simulink model "SVPWM"  (R2018a)
settings: Solver=FixedStepAuto  StartTime=0.0  StopTime=10.0  FixedStep=0.00001  RelTol=1e-3
libraries: simulink x1
settings Model: Creator=18236  LastModifiedBy=18236

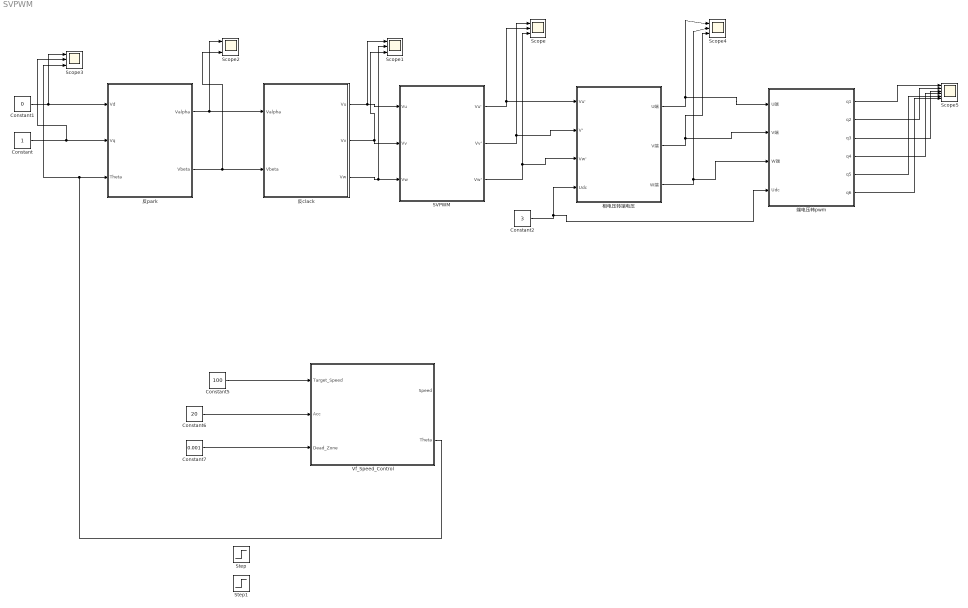
== system SVPWM ==
  Constant : Constant
  Constant1 : Constant  Value=0
  Constant2 : Constant  Value=3
  Constant5 : Constant  Value=100
  Constant6 : Constant  Value=20
  Constant7 : Constant  Value=0.001
  "SVPWM " : Subsystem
  Scope{,1..4} (5 alike) : Scope  NumInputPorts=3
  Scope5 : Scope  NumInputPorts=6
  Step : Step  Time=0  After=50  SampleTime=0
  Step1 : Step  Time=5  After=-100  SampleTime=0
  Vf_Speed_Control : Subsystem
  "反clack " : Subsystem
  "反park " : Subsystem
  "相电压转端电压 " : Subsystem
  端电压转pwm : Subsystem
  wires:
  Constant/1 -> Scope3/2, "反park "/2(Vq)
  Constant1/1 -> Scope3/1, "反park "/1("Vd ")
  "反park "/1("Valpha ") -> Scope2/1, "反clack "/1(Valpha)
  "反park "/2(Vbeta) -> Scope2/3, "反clack "/2(Vbeta)
  "反clack "/1(Vu) -> Scope1/1, "SVPWM "/1("Vu ")
  "反clack "/2(Vv) -> Scope1/3, "SVPWM "/2(Vv)
  "反clack "/3("Vw ") -> Scope1/2, "SVPWM "/3(Vw)
  "SVPWM "/1(Vu') -> "相电压转端电压 "/1(Vu'), Scope/2
  "SVPWM "/2(Vv') -> "相电压转端电压 "/2(V'), Scope/1
  "SVPWM "/3(Vw') -> "相电压转端电压 "/3(Vw'), Scope/3
  Constant2/1 -> 端电压转pwm/4(Udc), "相电压转端电压 "/4(Udc)
  "相电压转端电压 "/1(U端) -> 端电压转pwm/1(U端), Scope4/1
  "相电压转端电压 "/2(V端) -> 端电压转pwm/2(V端), Scope4/3
  "相电压转端电压 "/3(W端) -> 端电压转pwm/3(W端), Scope4/2
  端电压转pwm/1("q1 ") -> Scope5/1
  端电压转pwm/2(q2) -> Scope5/2
  端电压转pwm/3(q3) -> Scope5/3
  端电压转pwm/4(q4) -> Scope5/4
  端电压转pwm/5(q5) -> Scope5/5
  端电压转pwm/6(q6) -> Scope5/6
  Constant5/1 -> Vf_Speed_Control/1(Target_Speed)
  Constant6/1 -> Vf_Speed_Control/2(Acc)
  Constant7/1 -> Vf_Speed_Control/3(Dead_Zone)
  Vf_Speed_Control/2("Theta ") -> "反park "/3("Theta "), Scope3/3

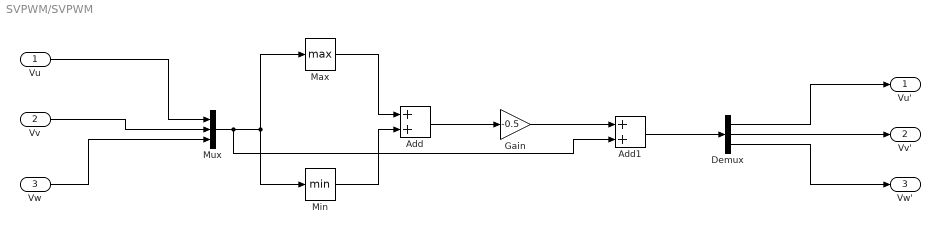
== system SVPWM/SVPWM  ==
  "Vu " : Inport
  Vv : Inport  Port=2
  Vw : Inport  Port=3
  Add : Sum
  Add1 : Sum
  Demux : Demux  Outputs=3
  Gain : Gain  Gain=-0.5
  Max : MinMax  Function=max
  Min : MinMax
  Mux : Mux  Inputs=3
  Vu' : Outport
  Vv' : Outport  Port=2
  Vw' : Outport  Port=3
  wires:
  "Vu "/1 -> Mux/1
  Vv/1 -> Mux/2
  Vw/1 -> Mux/3
  Mux/1 -> Add1/2, Min/1, Max/1
  Max/1 -> Add/1
  Min/1 -> Add/2
  Add/1 -> Gain/1
  Gain/1 -> Add1/1
  Add1/1 -> Demux/1
  Demux/1 -> Vu'/1
  Demux/2 -> Vv'/1
  Demux/3 -> Vw'/1

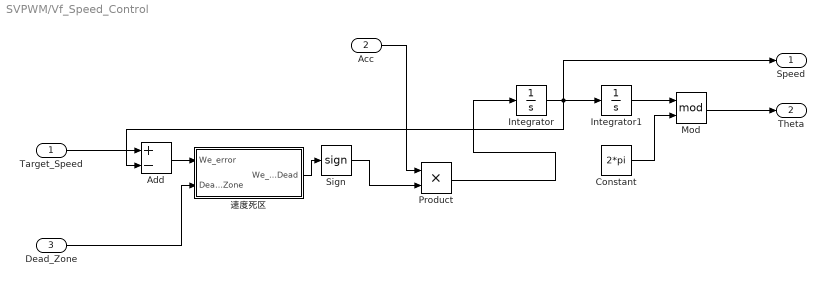
== system SVPWM/Vf_Speed_Control ==
  Target_Speed : Inport
  Acc : Inport  Port=2
  Dead_Zone : Inport  Port=3
  Add : Sum  Inputs=+-
  Constant : Constant  Value=2*pi
  Integrator : Integrator
  Integrator1 : Integrator
  Mod : Math  Operator=mod  SaturateOnIntegerOverflow=on
  Product : Product
  Sign : Signum
  "速度死区 " : MATLAB Function  TreatAsAtomicUnit=on
  Speed : Outport
  "Theta " : Outport  Port=2
  wires:
  Integrator/1 -> Add/2, Speed/1, Integrator1/1
  Integrator1/1 -> Mod/1
  Constant/1 -> Mod/2
  Mod/1 -> "Theta "/1
  Target_Speed/1 -> Add/1
  Add/1 -> "速度死区 "/1(We_error)
  Acc/1 -> Product/1
  Sign/1 -> Product/2
  Product/1 -> Integrator/1
  "速度死区 "/1(We_Error_Dead) -> Sign/1
  Dead_Zone/1 -> "速度死区 "/2(Dead_Zone)

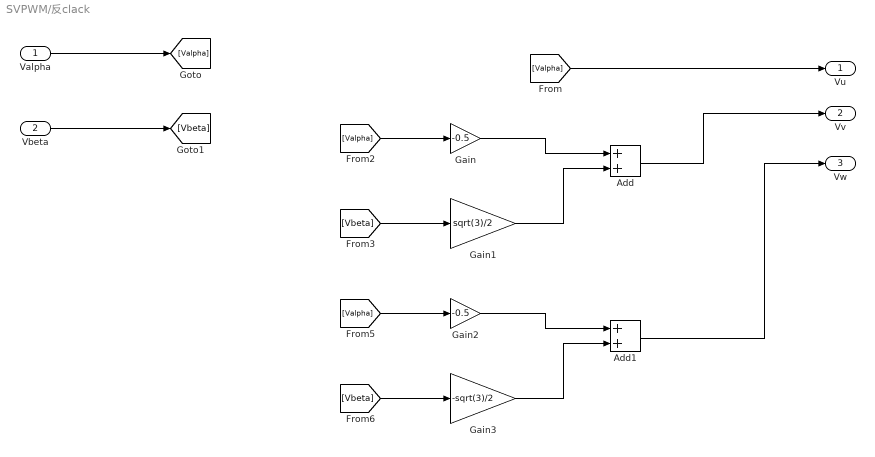
== system SVPWM/反clack  ==
  Valpha : Inport
  Vbeta : Inport  Port=2
  Add : Sum
  Add1 : Sum
  Gain : Gain  Gain=-0.5
  Gain1 : Gain  Gain=sqrt(3)/2
  Gain2 : Gain  Gain=-0.5
  Gain3 : Gain  Gain=-sqrt(3)/2
  Vu : Outport
  Vv : Outport  Port=2
  "Vw " : Outport  Port=3
  wires:
  Valpha/1 -> [Valpha]
  Vbeta/1 -> [Vbeta]
  [Valpha] -> Vu/1
  [Valpha] -> Gain/1
  [Vbeta] -> Gain1/1
  Gain/1 -> Add/1
  Gain1/1 -> Add/2
  Add/1 -> Vv/1
  [Valpha] -> Gain2/1
  [Vbeta] -> Gain3/1
  Gain2/1 -> Add1/1
  Gain3/1 -> Add1/2
  Add1/1 -> "Vw "/1

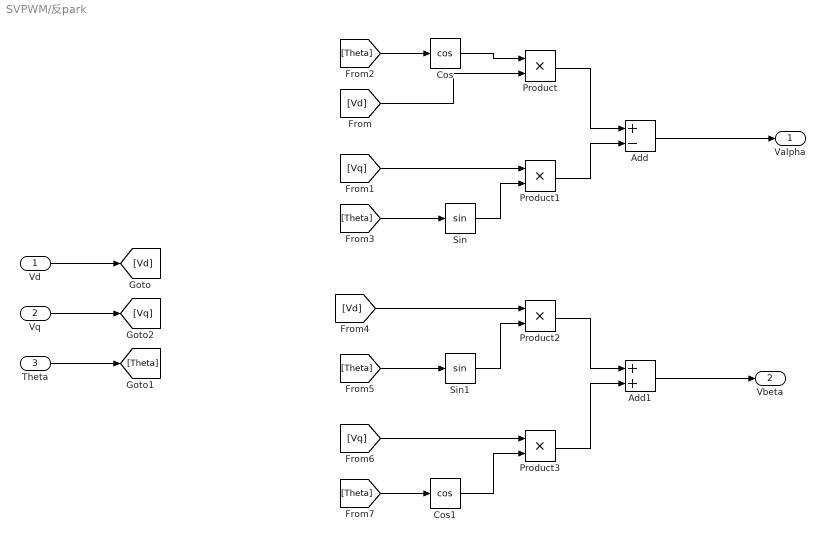
== system SVPWM/反park  ==
  "Vd " : Inport
  Vq : Inport  Port=2
  "Theta " : Inport  Port=3
  Add : Sum  Inputs=+-
  Add1 : Sum
  Cos : Trigonometry  Operator=cos
  Cos1 : Trigonometry  Operator=cos
  Product{,1..3} (4 alike) : Product
  Sin : Trigonometry
  Sin1 : Trigonometry
  "Valpha " : Outport
  Vbeta : Outport  Port=2
  wires:
  "Vd "/1 -> [Vd]
  "Theta "/1 -> [Theta]
  Vq/1 -> [Vq]
  [Theta] -> Cos/1
  Cos/1 -> Product/1
  [Vd] -> Product/2
  [Theta] -> Sin/1
  [Vq] -> Product1/1
  Sin/1 -> Product1/2
  Product/1 -> Add/1
  Product1/1 -> Add/2
  Add/1 -> "Valpha "/1
  [Theta] -> Sin1/1
  [Vd] -> Product2/1
  Sin1/1 -> Product2/2
  [Theta] -> Cos1/1
  [Vq] -> Product3/1
  Cos1/1 -> Product3/2
  Product2/1 -> Add1/1
  Product3/1 -> Add1/2
  Add1/1 -> Vbeta/1

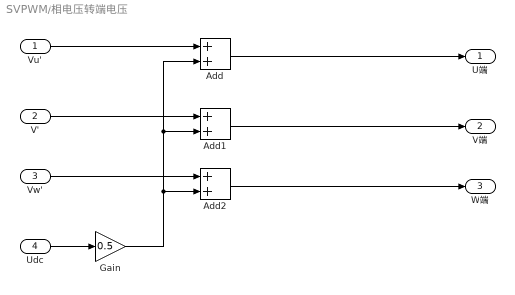
== system SVPWM/相电压转端电压  ==
  Vu' : Inport
  V' : Inport  Port=2
  Vw' : Inport  Port=3
  Udc : Inport  Port=4
  Add : Sum
  Add1 : Sum
  Add2 : Sum
  Gain : Gain  Gain=0.5
  U端 : Outport
  V端 : Outport  Port=2
  W端 : Outport  Port=3
  wires:
  Vu'/1 -> Add/1
  Udc/1 -> Gain/1
  Gain/1 -> Add/2, Add1/2, Add2/2
  Add/1 -> U端/1
  V'/1 -> Add1/1
  Add1/1 -> V端/1
  Vw'/1 -> Add2/1
  Add2/1 -> W端/1

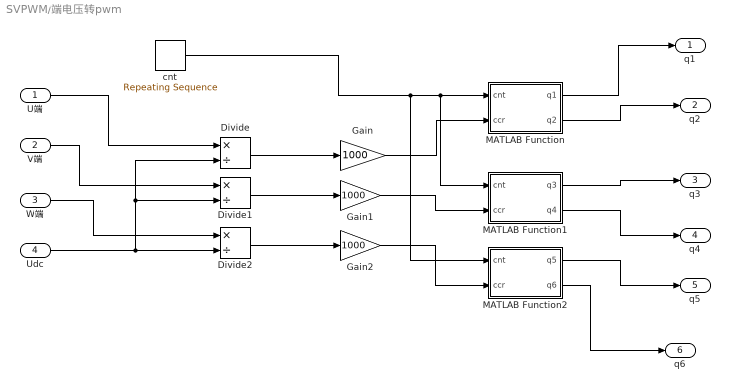
== system SVPWM/端电压转pwm ==
  U端 : Inport
  V端 : Inport  Port=2
  W端 : Inport  Port=3
  Udc : Inport  Port=4
  Divide : Product  Inputs=*/
  Divide1 : Product  Inputs=*/
  Divide2 : Product  Inputs=*/
  Gain : Gain  Gain=1000
  Gain1 : Gain  Gain=1000
  Gain2 : Gain  Gain=1000
  MATLAB Function : MATLAB Function  TreatAsAtomicUnit=on
  MATLAB Function1 : MATLAB Function  TreatAsAtomicUnit=on
  MATLAB Function2 : MATLAB Function  TreatAsAtomicUnit=on
  "cnt " : simulink/Sources/Repeating Sequence  rep_seq_t=[0 0.0005 0.001]  rep_seq_y=[0 1000 0]
  "q1 " : Outport
  q2 : Outport  Port=2
  q3 : Outport  Port=3
  q4 : Outport  Port=4
  q5 : Outport  Port=5
  q6 : Outport  Port=6
  wires:
  U端/1 -> Divide/1
  Udc/1 -> Divide2/2, Divide1/2, Divide/2
  Divide/1 -> Gain/1
  Divide1/1 -> Gain1/1
  Divide2/1 -> Gain2/1
  V端/1 -> Divide1/1
  W端/1 -> Divide2/1
  "cnt "/1 -> MATLAB Function2/1(cnt), MATLAB Function1/1(cnt), MATLAB Function/1(cnt)
  Gain/1 -> MATLAB Function/2(ccr)
  Gain1/1 -> MATLAB Function1/2(ccr)
  Gain2/1 -> MATLAB Function2/2(ccr)
  MATLAB Function/1(q1) -> "q1 "/1
  MATLAB Function/2(q2) -> q2/1
  MATLAB Function1/1(q3) -> q3/1
  MATLAB Function1/2(q4) -> q4/1
  MATLAB Function2/1(q5) -> q5/1
  MATLAB Function2/2(q6) -> q6/1

== matlab function SVPWM/端电压转pwm/MATLAB Function1 ==
  data: cnt input; q3 output; ccr input; q4 output
function [q3,q4] = fcn(cnt,ccr)

q3 = 0;
q4 = 0;
if(cnt < ccr)
    q3 = 1;
    q4 = 0;
elseif(cnt > ccr)
    q3 = 0;
    q4 = 1;
end


end

== matlab function SVPWM/端电压转pwm/MATLAB Function ==
  data: cnt input; q1 output; ccr input; q2 output
function [q1,q2] = fcn(cnt,ccr)

q1 = 0;
q2 = 0;
if(cnt < ccr)
    q1 = 1;
    q2 = 0;
elseif(cnt > ccr)
    q1 = 0;
    q2 = 1;
end


end

== matlab function SVPWM/端电压转pwm/MATLAB Function2 ==
  data: cnt input; q5 output; ccr input; q6 output
function [q5,q6] = fcn(cnt,ccr)

q5 = 0;
q6 = 0;
if(cnt < ccr)
    q5 = 1;
    q6 = 0;
elseif(cnt > ccr)
    q5 = 0;
    q6 = 1;
end


end

== matlab function SVPWM/Vf_Speed_Control/速度死区  ==
  data: We_error input; We_Error_Dead output; Dead_Zone input
function We_Error_Dead = fcn(We_error,Dead_Zone)

if(abs(We_error)<Dead_Zone)
    We_Error_Dead = 0;
else
    We_Error_Dead = We_error;
end
end
